simulink model "drone_nocontroller"  (R2026b)
settings: Solver=VariableStepAuto
settings Model: Creator=Miruna  LastModifiedBy=Miruna

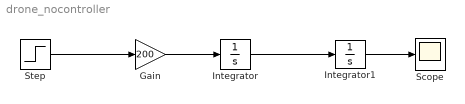
== system drone_nocontroller ==
  Gain : Gain  Gain=200
  Integrator : Integrator
  Integrator1 : Integrator
  Scope : Scope
      settings: ActiveDisplayYMinimum=-8.26023986838459  ActiveDisplayYMaximum=12.439592426168135
  Step : Step  FinalValue=0.001  SampleTime=0
  wires:
  Integrator/1 -> Integrator1/1
  Step/1 -> Gain/1
  Gain/1 -> Integrator/1
  Integrator1/1 -> Scope/1
